simulink model "comparison"  (R2025b)
settings: Solver=ode23tb  StartTime=0.0  StopTime=0.1  MaxStep=tc  RelTol=1e-3
values from neighbouring files (symbols this model uses):
  udc_1 = 500*kv    (= 1.03448275862)    [init.m]
  udc_2 = 750*kv    (= 1.55172413793)    [init.m]
  udc_lim = 600*kv    (= 1.24137931034)    [init.m]
libraries: fl_lib x20, nesl_utility x4, ee_lib x2, opamp x2
settings Model: Creator=ltnbda  LastModifiedBy=ltnbda
settings DataIOCC: SaveOutput=off  SignalLogging=off  DSMLogging=off  SaveTime=off  ReturnWorkspaceOutputs=off

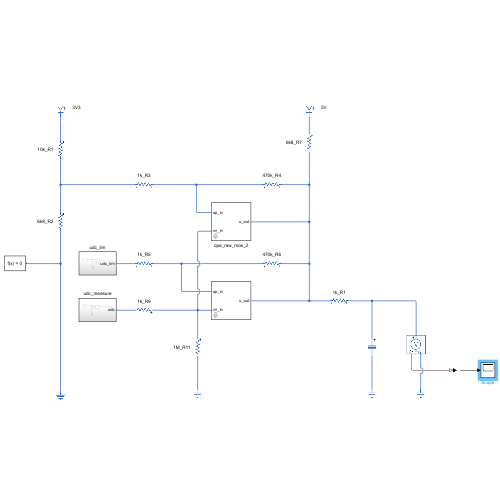
[thumbnail: Simulink's stored preview of the top-level diagram]
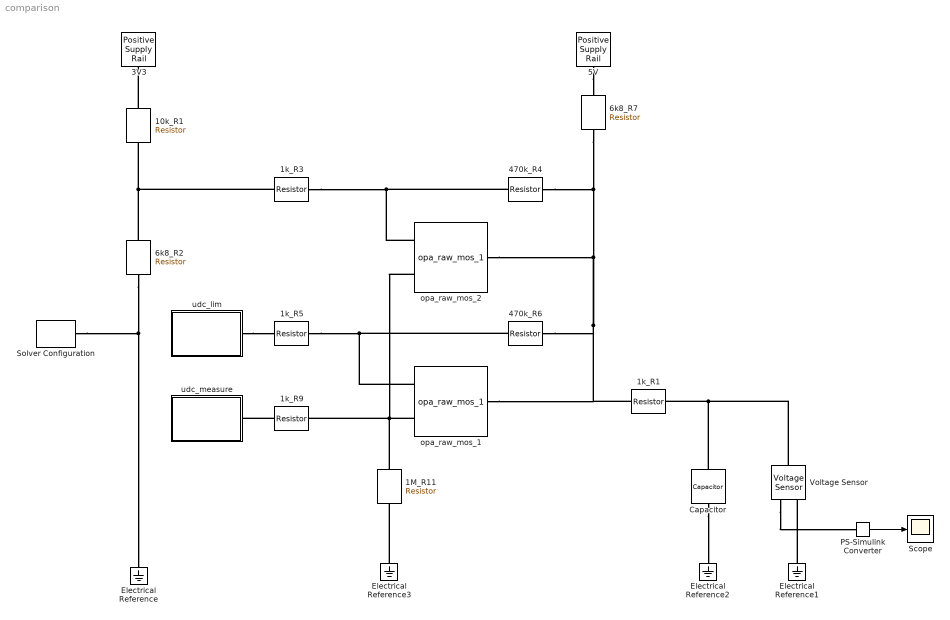
== system comparison ==
  10k_R1 : fl_lib/Electrical/Electrical Elements/Resistor  R=10e3 Ohm  i_specify=off  i_priority=None  i=0 A  i_nominal_specify=off  i_nominal_value=1  i_nominal_unit=A  v_specify=off  v_priority=None  v=0 V  v_nominal_specify=off  v_nominal_value=1  v_nominal_unit=V
  1M_R11 : fl_lib/Electrical/Electrical Elements/Resistor  R=1e6 Ohm  i_specify=off  i_priority=None  i=0 A  i_nominal_specify=off  i_nominal_value=1  i_nominal_unit=A  v_specify=off  v_priority=None  v=0 V  v_nominal_specify=off  v_nominal_value=1  v_nominal_unit=V
  1k_R{1,3,5,9} (4 alike) : fl_lib/Electrical/Electrical Elements/Resistor  R=1e3 Ohm  i_specify=off  i_priority=None  i=0 A  i_nominal_specify=off  i_nominal_value=1  i_nominal_unit=A  v_specify=off  v_priority=None  v=0 V  v_nominal_specify=off  v_nominal_value=1  v_nominal_unit=V
  3V3 : ee_lib/Sources/Positive Supply Rail  v0=3.3 V
      settings: InternalSimscapePortConfiguration="{\"Bottom\":[],\"Left\":[],\"Right\":[{\"id\":\"p\",\"label\":\"\",\"type\":\"foundation.electrical.electrical\"}],\"Top\":[]}"
  470k_R4 : fl_lib/Electrical/Electrical Elements/Resistor  R=470e3 Ohm  i_specify=off  i_priority=None  i=0 A  i_nominal_specify=off  i_nominal_value=1  i_nominal_unit=A  v_specify=off  v_priority=None  v=0 V  v_nominal_specify=off  v_nominal_value=1  v_nominal_unit=V
  470k_R6 : fl_lib/Electrical/Electrical Elements/Resistor  R=470e3 Ohm  i_specify=off  i_priority=None  i=0 A  i_nominal_specify=off  i_nominal_value=1  i_nominal_unit=A  v_specify=off  v_priority=None  v=0 V  v_nominal_specify=off  v_nominal_value=1  v_nominal_unit=V
  5V : ee_lib/Sources/Positive Supply Rail  v0=15 V
      settings: InternalSimscapePortConfiguration="{\"Bottom\":[],\"Left\":[],\"Right\":[{\"id\":\"p\",\"label\":\"\",\"type\":\"foundation.electrical.electrical\"}],\"Top\":[]}"
  6k8_R2 : fl_lib/Electrical/Electrical Elements/Resistor  R=6.8e3 Ohm  i_specify=off  i_priority=None  i=0 A  i_nominal_specify=off  i_nominal_value=1  i_nominal_unit=A  v_specify=off  v_priority=None  v=0 V  v_nominal_specify=off  v_nominal_value=1  v_nominal_unit=V
  6k8_R7 : fl_lib/Electrical/Electrical Elements/Resistor  R=6.8e3 Ohm  i_specify=off  i_priority=None  i=0 A  i_nominal_specify=off  i_nominal_value=1  i_nominal_unit=A  v_specify=off  v_priority=None  v=0 V  v_nominal_specify=off  v_nominal_value=1  v_nominal_unit=V
  Capacitor : fl_lib/Electrical/Electrical Elements/Capacitor  c=1e-6 F  r=1e-6 Ohm  g=0 1/Ohm  i_specify=off  i_priority=None  i=0 A  i_nominal_specify=off  i_nominal_value=1  i_nominal_unit=A  v_specify=off  v_priority=None  v=0 V  v_nominal_specify=off  v_nominal_value=1  v_nominal_unit=V  vc_specify=off  vc_priority=High  vc=0 V  vc_nominal_specify=off  vc_nominal_value=1  vc_nominal_unit=V
  Electrical Reference{,1..3} (4 alike) : fl_lib/Electrical/Electrical Elements/Electrical Reference
  PS-Simulink Converter : nesl_utility/PS-Simulink Converter  PhysicalDomain=network_engine_domain  SubClassName=ps_output  LeftPortType=input  RightPortType=output  PseudoPeriodic=off  Frequencies=[]  VectorFormat=inherit  Unit=inherit  AffineConversion=off
  Scope : Scope
      settings: ActiveDisplayYMinimum=-0.62309308953855269  ActiveDisplayYMaximum=5.6284840323879326
  Solver Configuration : nesl_utility/Solver Configuration  PhysicalDomain=network_engine_domain  SubClassName=solver  LeftPortType=input  RightPortType=generic  Tones=[]  Harmonics=[]  SimulateNoise=off  Profile=off  UseLocalSampling=off  EnableSwitchedLinearOptims=on  FrequencyDomain=off  UseCCode=off  RelTol=0.001  AbsTol=0.001  MinStep=1e-09  ToWorkspace=off  RevertToSquareIcSolve=off  NumHomotopyIterations=100  PhasorMode=off  PhasorModeNumHarmonics=1  ConsistencySolver=NEWTON_XTOL_AFTER_FTOL  IndexReductionMethod=DerivativeReplacement  DoDC=on  ResidualTolerance=1e-09  ConsistencyTolSource=GLOBAL  ConsistencyAbsTol=0.001  ConsistencyRelTol=0.001  ConsistencyTolFactor=0.001  UseLocalSolver=on  LocalSolverChoice=NE_BACKWARD_EULER_ADVANCER  ResolveIndetEquations=on  FunctionEvalNumThread=1  LocalSolverSampleTime=tc  DoFixedCost=on  MaxNonlinIter=5  MaxModeIter=2  ComputeImpulses=off  ImpulseIterations=2  LinearAlgebra=auto  LinearAlgebraNumThread=0  EquationFormulation=NE_TIME_EF  DelaysMemoryBudget=1024  AutomaticFiltering=on  FilteringTimeConstant=0.001  PartitionStorageMethod=AS_NEEDED  PartitionMemoryBudget=1024  PartitionMethod=ROBUST  MultibodyUseLocalSolver=off  MultibodyLocalSolverChoice=ODE1  MultibodyLocalSolverSampleTime=0.001
  Voltage Sensor : fl_lib/Electrical/Electrical Sensors/Voltage Sensor
  opa_raw_mos_1 : opamp/opa_raw_mos_1  u_dd=5  u_ss=0  Rbias=300
  opa_raw_mos_2 : opamp/opa_raw_mos_1  u_dd=5  u_ss=0  Rbias=300
  udc_lim : Subsystem
  udc_measure : Subsystem
  wires:
  PS-Simulink Converter/1 -> Scope/1
  connections:
  10k_R1/LConn1 -- 3V3/RConn1
  6k8_R2/LConn1 -- 1k_R3/RConn1 -- 10k_R1/RConn1
  6k8_R2/RConn1 -- Electrical Reference/LConn1 -- Solver Configuration/RConn1
  1k_R3/LConn1 -- opa_raw_mos_2/LConn1 -- 470k_R4/RConn1
  470k_R6/RConn1 -- opa_raw_mos_1/LConn1 -- 1k_R5/LConn1
  1k_R9/RConn1 -- udc_measure/LConn1
  udc_lim/LConn1 -- 1k_R5/RConn1
  Electrical Reference1/LConn1 -- Voltage Sensor/RConn2
  Voltage Sensor/RConn1 -- PS-Simulink Converter/LConn1
  5V/RConn1 -- 6k8_R7/LConn1
  Capacitor/RConn1 -- Electrical Reference2/LConn1
  1M_R11/LConn1 -- opa_raw_mos_2/LConn2 -- opa_raw_mos_1/LConn2 -- 1k_R9/LConn1
  470k_R4/LConn1 -- 6k8_R7/RConn1 -- opa_raw_mos_2/RConn1 -- opa_raw_mos_1/RConn1 -- 1k_R1/RConn1 -- 470k_R6/LConn1
  Electrical Reference3/LConn1 -- 1M_R11/RConn1
  Voltage Sensor/LConn1 -- Capacitor/LConn1 -- 1k_R1/LConn1

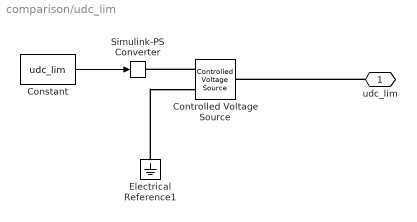
== system comparison/udc_lim ==
  Constant : Constant  Value=udc_lim
  Controlled Voltage Source : fl_lib/Electrical/Electrical Sources/Controlled Voltage Source
  Electrical Reference1 : fl_lib/Electrical/Electrical Elements/Electrical Reference
  Simulink-PS Converter : nesl_utility/Simulink-PS Converter  PhysicalDomain=network_engine_domain  SubClassName=ps_input  LeftPortType=input  RightPortType=output  PseudoPeriodic=off  Frequencies=[]  NoiseDistribution=none  NoiseParameters=[]  Unit=V  AffineConversion=off  FilteringAndDerivatives=provide  SimscapeFilterOrder=1  InputFilterTimeConstant=0.001  UdotUserProvided=0
  udc_lim : PMIOPort  Side=Left
  wires:
  Constant/1 -> Simulink-PS Converter/1
  connections:
  Controlled Voltage Source/RConn1 -- Simulink-PS Converter/RConn1
  Electrical Reference1/LConn1 -- Controlled Voltage Source/RConn2
  udc_lim/RConn1 -- Controlled Voltage Source/LConn1

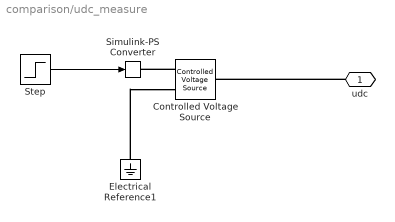
== system comparison/udc_measure ==
  Controlled Voltage Source : fl_lib/Electrical/Electrical Sources/Controlled Voltage Source
  Electrical Reference1 : fl_lib/Electrical/Electrical Elements/Electrical Reference
  Simulink-PS Converter : nesl_utility/Simulink-PS Converter  PhysicalDomain=network_engine_domain  SubClassName=ps_input  LeftPortType=input  RightPortType=output  PseudoPeriodic=off  Frequencies=[]  NoiseDistribution=none  NoiseParameters=[]  Unit=V  AffineConversion=off  FilteringAndDerivatives=provide  SimscapeFilterOrder=1  InputFilterTimeConstant=0.001  UdotUserProvided=0
  Step : Step  Time=0.05  Before=udc_1  After=udc_2  SampleTime=0
  udc : PMIOPort  Side=Left
  wires:
  Step/1 -> Simulink-PS Converter/1
  connections:
  udc/RConn1 -- Controlled Voltage Source/LConn1
  Electrical Reference1/LConn1 -- Controlled Voltage Source/RConn2
  Controlled Voltage Source/RConn1 -- Simulink-PS Converter/RConn1
